simulink model "acf_sea_pad_research_20261006"  (R2026b)
settings: Solver=ode4  StopTime=p.stopTime  FixedStep=2.5000000000000002e-06
model workspace (MAT data in the model file):
  p.dt = 2.5e-06
  p.controlStep = 0.0001
  p.stopTime = 2
  p.mA = 1.5
  p.mB = 0.6
  p.mS = 2
  p.gAxis = 6.00484126643e-16
  p.Fref = 5
  p.kUpper = 20000
  p.kCell = 64000000
  p.sea = 0
  p.mNut = 0.075
  p.kSea = 5000
  p.cSea = 0
  p.preload = 0
  p.ell = 0.000795774715459
  p.Jtotal = 7.04e-06
  p.Kf = 24.4
  p.Kt = 0.0758
  p.Ke = 0.0758
  p.R = 8.896
  p.L = 0.004
  p.Imax = 3.5
  p.Vmax = 32
  p.currentTau = 5e-05
  p.guideCoulomb = 0.2
  p.guideViscous = 2
  p.guideSmooth = 0.001
  p.shaftCoulomb = 0.001
  p.shaftViscous = 1e-06
  p.shaftSmooth = 1
  p.kPad = 100000
  p.cPad = 150
  p.padDiameter = 0.077
  p.stripCount = 61
  p.bumpTime = 0.8
  p.bumpHeight = 0.001
  p.bumpWidth = 0.01
  p.scanSpeed = 0.1
  p.toolTravelLimit = 0.0125
  p.nutTravelLimit = 0.05
  p.springTravelLimit = 0.017
  p.padCompressionLimit = 0.0025
  p.enableStops = 1
  p.offsets = [-0.037868852459; -0.036606557377; -0.0353442622951; -0.0340819672131; -0.0328196721311; -0.0315573770492; -0.0302950819672; -0.0290327868852; -0.0277704918033; -0.0265081967213; -0.0252459016393; -0.0239836065574; -0.0227213114754; -0.0214590163934; -0.0201967213115; -0.0189344262295; -0.0176721311475; -0.0164098360656; -0.0151475409836; -0.0138852459016; -0.0126229508197; -0.0113606557377; -0.0100983606557; -0.00883606557377; -0.0075737704918; -0.00631147540984; -0.00504918032787; -0.0037868852459; -0.00252459016393; -0.00126229508197; 0; 0.00126229508197; 0.00252459016393; 0.0037868852459; 0.00504918032787; 0.00631147540984; 0.0075737704918; 0.00883606557377; 0.0100983606557; 0.0113606557377; 0.0126229508197; 0.0138852459016; 0.0151475409836; 0.0164098360656; 0.0176721311475; 0.0189344262295; 0.0201967213115; 0.0214590163934; 0.0227213114754; 0.0239836065574; 0.0252459016393; 0.0265081967213; 0.0277704918033; 0.0290327868852; 0.0302950819672; 0.0315573770492; 0.0328196721311; 0.0340819672131; 0.0353442622951; 0.036606557377; 0.037868852459]
  p.weights = [0.00354573794381 0.00643311477612 0.00826104427713 0.00969909185977 0.0109056081557 0.0119516353177 0.0128765964345 0.0137051352446 0.0144538976089 0.0151347586863 0.015756541158 0.0163260077674 0.0168484714702 0.0173281894083 0.0177686276348 0.0181726449385 0.0185426240574 0.0188805675467 0.0191881692235 0.0194668683153 0.0197178910871 0.0199422832222 0.0201409352482 0.020314602639 0.0204639217736 0.0205894226123 0.0206915387269 0.0207706151559 0.0208269144326 0.0208606210401 0.0208718444751 0.0208606210401 0.0208269144326 0.0207706151559 0.0206915387269 0.0205894226123 0.0204639217736 0.020314602639 0.0201409352482 0.0199422832222 0.0197178910871 0.0194668683153 0.0191881692235 0.0188805675467 0.0185426240574 0.0181726449385 0.0177686276348 0.0173281894083 0.0168484714702 0.0163260077674 0.015756541158 0.0151347586863 0.0144538976089 0.0137051352446 0.0128765964345 0.0119516353177 0.0109056081557 0.00969909185977 0.00826104427713 0.00643311477612 0.00354573794381]
  p.centerWeight = [0 0 0 0 0 0 0 0 0 0 0 0 0 0 0 0 0 0 0 0 0 0 0 0 0 0 0 0 0 0 1 0 0 0 0 0 0 0 0 0 0 0 0 0 0 0 0 0 0 0 0 0 0 0 0 0 0 0 0 0 0]
  p.rigidPoint = 0
  p.initial = [0.00025 0 -5.0078125e-05 0 -5e-05 0 0 0 0.204918032787]
  p.massInverse = [0.635123304033  0.00425605136463; 0.00425605136463  0.0893770786572]
  replayInputs = [0 0.0001 0.0002 0.0003 0.0004 0.0005 0.0006 0.0007 0.0008 0.0009 0.001 0.0011 ... (60003 elements, 20001x3)]
libraries: simulink x1
(part 1 of 2)
settings Model: Creator=tommie  LastModifiedBy=tommie
settings DataIOCC: ExternalInput=replayInputs  LoadExternalInput=on  SignalLogging=off

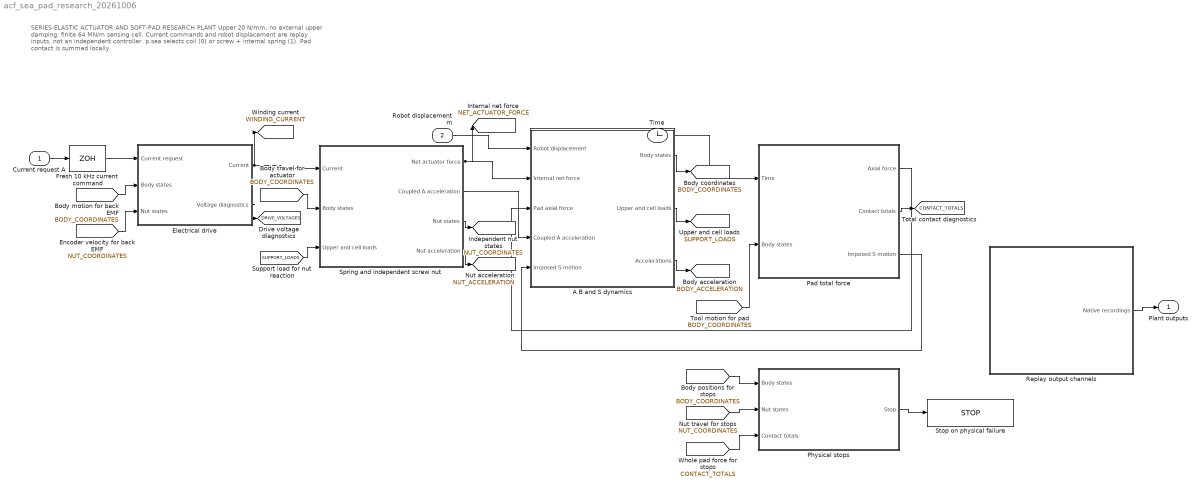
== system acf_sea_pad_research_20261006 ==
  note: SERIES-ELASTIC ACTUATOR AND SOFT-PAD RESEARCH PLANT
      | Upper 20 N/mm, no external upper damping; finite 64 MN/m sensing cell.
      | Current commands and robot displacement are replay inputs, not an independent controller.
      | p.sea selects coil (0) or screw + internal spring (1). Pad contact is summed locally.
  Current request A : Inport
  Robot displacement m : Inport  Port=2
  A B and S dynamics : Subsystem
  Electrical drive : Subsystem
  Fresh 10 kHz current command : ZeroOrderHold  SampleTime=p.controlStep
  Pad total force : Subsystem
  Physical stops : Subsystem
  Replay output channels : Subsystem
  Spring and independent screw nut : Subsystem
  Stop on physical failure : Stop
  Time : Clock
  Plant outputs : Outport
  tag scope: BODY_ACCELERATION=global, BODY_COORDINATES=global, CONTACT_TOTALS=global, DRIVE_VOLTAGES=global, NET_ACTUATOR_FORCE=global, NUT_ACCELERATION=global, NUT_COORDINATES=global, SUPPORT_LOADS=global, WINDING_CURRENT=global
  wires:
  Current request A/1 -> Fresh 10 kHz current command/1
  Fresh 10 kHz current command/1 -> Electrical drive/1(Current request)
  Electrical drive/1(Current) -> Spring and independent screw nut/1(Current), [WINDING_CURRENT]
  Robot displacement m/1 -> A B and S dynamics/1(Robot displacement)
  Spring and independent screw nut/1(Net actuator force) -> A B and S dynamics/2(Internal net force), [NET_ACTUATOR_FORCE]
  Pad total force/1(Axial force) -> A B and S dynamics/3(Pad axial force)
  Spring and independent screw nut/2(Coupled A acceleration) -> A B and S dynamics/4(Coupled A acceleration)
  Pad total force/3(Imposed S motion) -> A B and S dynamics/5(Imposed S motion)
  Time/1 -> Pad total force/1(Time)
  A B and S dynamics/1(Body states) -> [BODY_COORDINATES]
  Spring and independent screw nut/3(Nut states) -> [NUT_COORDINATES]
  A B and S dynamics/2(Upper and cell loads) -> [SUPPORT_LOADS]
  A B and S dynamics/3(Accelerations) -> [BODY_ACCELERATION]
  Electrical drive/2(Voltage diagnostics) -> [DRIVE_VOLTAGES]
  Pad total force/2(Contact totals) -> [CONTACT_TOTALS]
  Spring and independent screw nut/4(Nut acceleration) -> [NUT_ACCELERATION]
  [BODY_COORDINATES] -> Electrical drive/2(Body states)
  [NUT_COORDINATES] -> Electrical drive/3(Nut states)
  [BODY_COORDINATES] -> Spring and independent screw nut/2(Body states)
  [SUPPORT_LOADS] -> Spring and independent screw nut/3(Upper and cell loads)
  [BODY_COORDINATES] -> Pad total force/2(Body states)
  [BODY_COORDINATES] -> Physical stops/1(Body states)
  [NUT_COORDINATES] -> Physical stops/2(Nut states)
  [CONTACT_TOTALS] -> Physical stops/3(Contact totals)
  Physical stops/1(Stop) -> Stop on physical failure/1
  Replay output channels/1(Native recordings) -> Plant outputs/1
